simulink model "commhdlQPSKTxRxLoopback"  (R2025b)
settings: Solver=FixedStepDiscrete  StartTime=0.0  StopTime=stopTime  RelTol=1e-3
PostLoadFcn:
  | hScopeConfig = get_param([gcs '/Receiver/QPSK Rx/Frequency and Time Synchronizer/Symbol Synchronizer/No HDL/QPSK Receiver Eye Diagram'],'ScopeConfiguration');
  | 
  | hScopeConfig.OpenAtSimulationStart = false;
  | hScopeConfig.Visible = false;
  | SamplesPerSymbol = 4;
  | %UpsamplesRx = 1;
  | clear hScopeConfig
InitFcn:
  | commhdlQPSKTxRxModelInit;
  | % Rate bridge: ADRV9002/Jupiter radio runs at 15.36 MHz = 2x the 7.68 MHz
  | % (4 samples/symbol @ Rsym=1.92 MHz) the QPSK Rx requires. The deployed
  | % Receiver must downsample the ADC stream by 2. UpsamplesRx=1 fed the QPSK
  | % Rx 8 sps (2x-upsampled) and broke symbol sync / the loopback bit check.
  | UpsamplesRx = 1;   %% T8 RATE FIX: rail 15.36e6 == ADC bus rate,
  | %% no ingress decimation (was 2 when the rail sat on the 7.68e6 rung)
  | UpsamplesTx = 1;
  | clear simTimingOffset;
StopFcn:
  | if exist('simTimingOffset','var')
  |   disp('Simulation completed');
  |   %QPSKTxRxVerification;
  | end
undefined symbols (not defined in the file or in its folder): Add, Config, fsym, randsrc, RandStream, Rsym, Shift
libraries: hdlsllib x141, simulink x43, dspsigops x34, dsphdlfiltering2 x6, dsphdlsigops2 x4, dsphdlmathfun2 x4, commdigbbndpm3 x4, dspmlti4 x2, commchan3 x1, commrflib2 x1, commcnvcod2 x1
(part 8 of 8)

== matlab function commhdlQPSKTxRxLoopback/TxRxComposite/Receiver/QPSK Rx/Frequency and Time Synchronizer/Coarse Frequency Compensator/CFO step change detector/LGMux_cfo_threshold ==
  data: axi input; firePos output; x input; fireNeg output; nz output
function [firePos, fireNeg, nz] = cfo_threshold_mux(axi, x)
%#codegen
nz = axi ~= uint32(0);
si = bitsliceget(axi, 22, 1);
thr = reinterpretcast(si, numerictype(1, 22, 21));
firePos = x > thr;
fireNeg = x < (-thr);
end

== matlab function commhdlQPSKTxRxLoopback/TxRxComposite/FrameStatChecksum ==
  data: word input uint64; chk output uint16; wordTog input boolean; strobe input boolean
function chk = frameStatChecksum(word, wordTog, strobe)
%#codegen
% 16-bit running checksum over the delivered RX 64-bit words. On each emitted
% word (wordTog change), the eight bytes of the word are added into a 16-bit
% modular accumulator. chk is COMBINATIONAL (= the accumulated sum of every
% word delivered in the frame completed as of this cycle) so FrameStatProbe,
% latching chk on the SAME strobe edge, captures THIS frame -- no register-to-
% register race / off-by-one (see FRAMESTAT_NOTES.md). Host mirror: for each
% received 64-bit word, add its 8 bytes mod 2^16.
persistent acc prevTog prevStr
if isempty(acc)
    acc = uint16(0); prevTog = false; prevStr = false;
end
chk = acc;
strobeEdge = strobe && ~prevStr;
prevStr = strobe;
if strobeEdge
    acc = uint16(0);
end
if logical(wordTog) ~= prevTog
    s = uint32(0);
    for bpos = 0:8:56
        s = s + uint32(bitand(bitshift(word, -bpos), uint64(255)));
    end
    acc = uint16(mod(uint32(acc) + s, uint32(65536)));
end
prevTog = logical(wordTog);

== matlab function commhdlQPSKTxRxLoopback/Transmitter/QPSK Tx/Bit Packetizer/Data Bits FIFO/RAM Frame Status Indicator ==
  data: push input; out output; pop input; dataBitsPerPacket parameter
function out = fcn(push,pop,dataBitsPerPacket)

   persistent pushCount popCount frameCount;
   if isempty(pushCount)
       pushCount = fi(0,0,nextpow2(dataBitsPerPacket),0,hdlfimath);
       frameCount = fi(0,0,2,0,hdlfimath);
       popCount = fi(0,0,nextpow2(dataBitsPerPacket),0,hdlfimath);
   end
   
   if (pushCount == dataBitsPerPacket-1) && push
       frameCount(:) = frameCount + 1;
   end
   if (popCount == dataBitsPerPacket-1) && pop
       frameCount(:) = frameCount - 1;
   end

   if push
       if pushCount == dataBitsPerPacket - 1
           pushCount(:) = 0;
       else
           pushCount(:) = pushCount + 1;
       end
   end

   if pop 
       if popCount == dataBitsPerPacket - 1
           popCount(:) = 0;
       else
           popCount(:) = popCount + 1;
       end
   end

   out = frameCount;

end

== matlab function commhdlQPSKTxRxLoopback/TxRxComposite/FrameStatProbe ==
  data: pktCnt input uint32; rec output uint64; rstcsCnt input uint32; runMax input uint32; adcFor input uint32; cfcEst input uint32; chk input uint16; strobe input boolean; push output boolean
function [rec, push] = frameStatProbe(pktCnt, rstcsCnt, runMax, adcFor, cfcEst, chk, strobe)
%#codegen
% Latch the 64-bit per-frame status record at the frame strobe. Bit layout:
%   [7:0] frame_seq [8] cs_reset [11] sync_low [23:16] corr [31:24] agc
%   [47:32] cfc [63:48] checksum. See FRAMESTAT_NOTES.md.
persistent rec_r prevRst prevStr
if isempty(rec_r)
    rec_r = uint64(0); prevRst = uint32(0); prevStr = false;
end
push = false;
% latch once per frame on the strobe rising edge (recStart pulse-or-hold safe)
strobeEdge = strobe && ~prevStr;
prevStr = strobe;
if strobeEdge
    frame_seq = uint64(bitand(pktCnt, uint32(255)));
    cs_reset  = uint64(rstcsCnt ~= prevRst);
    % corr_strength = MSB position (0..32) of the runningMax SI
    corrq = uint32(0);
    for k = 0:31
        if bitshift(runMax, -k) ~= uint32(0)
            corrq = uint32(k + 1);
        end
    end
    sync_low = uint64(corrq < uint32(20));
    corr8 = uint64(bitand(corrq, uint32(255)));
    agc8  = uint64(bitand(bitshift(adcFor, -24), uint32(255)));
    cfc16 = uint64(bitand(bitshift(cfcEst, -5), uint32(65535)));
    chk16 = uint64(chk);
    rec_r = bitor(bitor(bitor(bitor(bitor(bitor( ...
        frame_seq, ...
        bitshift(cs_reset, 8)), ...
        bitshift(sync_low, 11)), ...
        bitshift(corr8, 16)), ...
        bitshift(agc8, 24)), ...
        bitshift(cfc16, 32)), ...
        bitshift(chk16, 48));
    prevRst = rstcsCnt;
    push = true;
end
rec = rec_r;

== matlab function commhdlQPSKTxRxLoopback/TxRxComposite/FrameStatFifo ==
  data: rec input uint64; headLo output uint32; push input boolean; popTok input uint32; headHi output uint32; stat output uint32
function [headLo, headHi, stat] = frameStatFifo(rec, push, popTok)
%#codegen
% 64-deep record FIFO. HEAD = mem(rd). Host: read 0x1D0 (lo), 0x1D4 (hi),
% then write a changed token to 0x1DC to advance. STAT(0x1D8) =
% {ovf[31:16] | level[15:0]}. Drop-newest on full.
persistent mem wr rd ovfCnt prevPop
if isempty(wr)
    mem = zeros(64,1,'uint64'); wr = uint16(0); rd = uint16(0);
    ovfCnt = uint16(0); prevPop = uint32(0);
end
if push
    nxt = uint16(mod(uint32(wr) + 1, 64));
    if nxt == rd
        if ovfCnt < uint16(65535), ovfCnt = ovfCnt + uint16(1); end
    else
        mem(uint32(wr)+1) = rec;
        wr = nxt;
    end
end
if popTok ~= prevPop
    if wr ~= rd, rd = uint16(mod(uint32(rd) + 1, 64)); end
end
prevPop = popTok;
head = mem(uint32(rd)+1);
headLo = uint32(bitand(head, uint64(4294967295)));
headHi = uint32(bitshift(head, -32));
level  = uint32(mod(uint32(wr) - uint32(rd) + 64, 64));
stat   = bitor(bitshift(uint32(ovfCnt), 16), level);

== matlab function commhdlQPSKTxRxLoopback/TxRxComposite/FrameStatWordCnt ==
  data: vld input boolean; cnt output uint32; rdy input boolean
function cnt = frameStatWordCnt(vld, rdy)
%#codegen
% free-running 32-bit accepted-word counter (byte_rx_valid && byte_rx_ready).
% Wraps mod 2^32 (uint32 native wrap is not guaranteed saturation-free in
% MLFB codegen defaults, so wrap explicitly).
persistent c
if isempty(c)
    c = uint32(0);
end
cnt = c;
if vld && rdy
    if c == uint32(4294967295)
        c = uint32(0);
    else
        c = c + uint32(1);
    end
end

== matlab function commhdlQPSKTxRxLoopback/Receiver/QPSK Rx/Frequency and Time Synchronizer/Packet Controller/sample discard controller ==
  data: dataIn input; validIn input; dataOut output; startIn input; endIn input; startOut output; endOut output; validOut output
function [dataOut,startOut,endOut,validOut] = controller(dataIn,validIn,startIn,endIn)
%#codegen

   persistent active dataOutReg validOutReg startOutReg endOutReg;
   if isempty(active)
      active  = false;
      dataOutReg = cast(0,'like',dataIn);
      validOutReg = false;
      startOutReg = false;
      endOutReg = false;
   end
   
   dataOut = dataOutReg;
   validOut = validOutReg;
   startOut = startOutReg;
   endOut = endOutReg;
   
   startOutReg = startIn;
   endOutReg = endIn;
   
   if startIn
       active = true;
   end
   
   if active
       dataOutReg(:) = dataIn;
       validOutReg = validIn;
   else
       dataOutReg(:) = 0;
       validOutReg = false;
   end
   
   if endIn
       if active 
           endOutReg = true;
       else
           endOutReg = false;
       end
       active = false;
   end
end

== matlab function commhdlQPSKTxRxLoopback/Receiver/QPSK Rx/Frequency and Time Synchronizer/Symbol Synchronizer/Interpolation Control ==
  data: mu output; Delta input; Underflow output
function [mu,Underflow] = Interpolation_ctrl(Delta)
% Implementation of modulo-1 counter for interpolation control listed in
% Figure 8.4.19 of "Digital Communications - A Discrete-Time Approach"
% by Michael Rice. See design details in Chapter 8.4.3 of the same book.
% 
% Input:
%   Delta - Loop filter output. If loop is in lock, delta would be small
% Output:
%   Underflow - Indicator of counter underflow. This is the strobe signal
%               for downstream processing
%   mu - Difference between actual sampling instant and the optimal instant,
%        between zero and one
%#codegen

% countReg - Counter value delayed by 1 sample
% muReg - The estimated timing error normalized by half QPSK symbols

   mask = fi(1-2^(-10),1,11,10);
   
   persistent countReg underflowReg muReg;
   if isempty(countReg)
       countReg  = fi(0,1,11,10);
       muReg = fi(0,1,11,10);
       underflowReg = false;
   end
   
   
   Underflow = underflowReg;
   mu = muReg;   
   
   
      % T8.4 anti-wedge clamp: if Delta <= -0.125 the decrementing counter
   % never underflows (strobes stop FOREVER -- Class-4 wedge / Class-1
   % episode mechanism; see tb_timing_wedge.v). Bound Delta so the
   % counter always decrements by >= 1 LSB.
   wlim = fi(255/1024,1,11,10);
   if Delta > wlim
       Delta = wlim;
   elseif Delta < -wlim
       Delta = fi(-255/1024,1,11,10);
   end
   counter = bitand(mask,countReg)-Delta-fi(0.25,1,11,10); % decrementing counter
   
   % if countReg is a nonnegative number,
   % then mod(countReg,1) equals the fractional part of countReg
   if counter < 0
       underflowReg = true;
       muReg = bitshift(bitand(mask,countReg),2);
       countReg = fi(counter+1,1,11,10);% create underflow to counter
   else
       underflowReg = false;
       countReg = fi(counter,1,11,10);
   end
   


end

== matlab function commhdlQPSKTxRxLoopback/Receiver/QPSK Rx/Frequency and Time Synchronizer/Preamble Detector/Correlator/ThresholdLimiter ==
  settings: fimath=hdlfimath
  data: x input; y output
function y = applyLowerLimit(x)
    % Apply a lower limit to the threshold.
    %#codegen
    
    % Threshold is computed by summing across 63 samples.
    % Set lower limit to be equivalent of all 63 samples
    % having their LSB set to 1 and all others set to 0. 
    lowerLimit = cast(0.01, 'like', x);
    
    if x < lowerLimit
        y = lowerLimit;
    else
        y = x;
    end
end

== matlab function commhdlQPSKTxRxLoopback/Transmitter/Input Data/Message Generator/MATLAB Function ==
  data: enable input; reset input; out output; start output; stop output; valid output; count_out output; msg_count_out output
function [out, start, stop, valid, count_out, msg_count_out] = msggen(enable, reset)

persistent indexCount;
persistent toggle;
persistent msgCount;
persistent msgCountAll;
persistent msgCountBitIndex;

if isempty(indexCount) || isempty(toggle) || isempty(msgCount) || isempty(msgCountBitIndex) || isempty(msgCountAll)
    indexCount = uint32(0);
    msgCount = uint32(1);
    msgCountAll = uint32(1);
    msgCountBitIndex = uint8(0);
    toggle = false;
end

%% Constants
strAscii = dec2bin('ADI Hello World', 8);
msgarray = reshape(strAscii', [1, numel(strAscii)]);
msgbits = logical(msgarray - 48);
msgbitsLen = length(msgbits);

fullMessageLen = uint32(2240-1); % Need the -1 to eat the feedback delay

% Bit counter
% N = 8;% 8-bit counter
% mask = uint32(2^N - 1);
% for k = 1:300
%     msgCount = bitand(msgCount + uint32(1), mask);   % wraps 255 -> 0
% end

%% Logic
if enable && ~reset
    % Set out data
    if indexCount < msgbitsLen % Insert msg
        out = msgbits(indexCount + 1);
        msgCountBitIndex = uint8(0);
    else % Zero padding: varying filler (counter digit + toggle bits)
        % caused periodic false-lock error bursts in the deployed BIST;
        % zero-padded payload matches the verified host golden structure.
        out = false;
        msgCountBitIndex = uint8(0);
    end

    % Flags
    start = indexCount == uint32(0);
    stop = indexCount == fullMessageLen;
    valid = true;

    % Counters
    if fullMessageLen == indexCount
        if msgCount >= 9
            msgCount = uint32(1);
        else
            msgCount = msgCount +  1;
            msgCountAll = msgCountAll + 1;
        end
    end
    if indexCount <= fullMessageLen
        indexCount = indexCount + 1;
    end

else % Enable == false

    if reset
        indexCount = uint32(0);
        % msgCount = uint32(0);
        msgCountBitIndex = uint8(0);
        toggle = false;
    end
    out = false;
    start = false;
    stop = false;
    valid = false;
end

if isempty(indexCount)
    count_out = uint32(0);
else
    count_out = indexCount;
end

msg_count_out = msgCountAll;
